simulink model "chaine_texte"  (R2023b)
settings: Solver=FixedStepDiscrete  StartTime=0.0  StopTime=(N/4 - 1)*4*Tb  FixedStep=4*Tb  RelTol=1e-3
values from neighbouring files (symbols this model uses):
  A = P.A    [parametres.m]    (also in partie2_1.m; partie2_5_q10.m = numel(unique(msg)); partie2_5_q11.m = numel(unique(seq)))
  Ac = A * sqrt(4/7)    [creer_chaine_hamming.m]
  graine = P.graine    [parametres.m]    (also in parametres_perso.m = mod(sum(c .* (1:numel(c)) * 31) + 7 * numel(c), 2^31 - 1); partie2_1.m)
  L = P.L    [parametres.m]    (also in partie2_1.m)
  sig2 = N0 * L / (2*Tb)    [parametres.m]    (also in partie3_q12.m = A^2 * L / (2 * 10^(EbN0dB/10)))
  Tb = 1    [parametres.m]    (also in partie2_1.m)
libraries: simulink x2
settings Model: Creator=e2507477  LastModifiedBy=e2507477

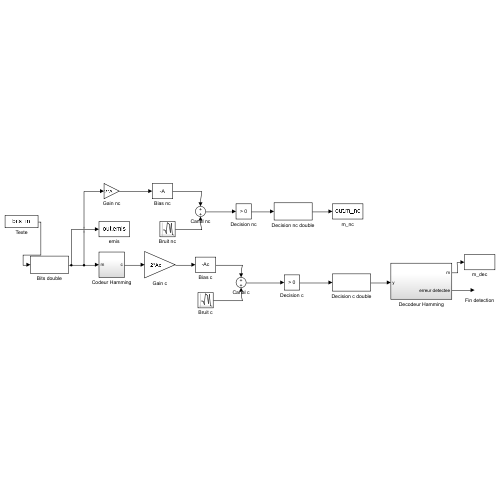
[thumbnail: Simulink's stored preview of the top-level diagram]
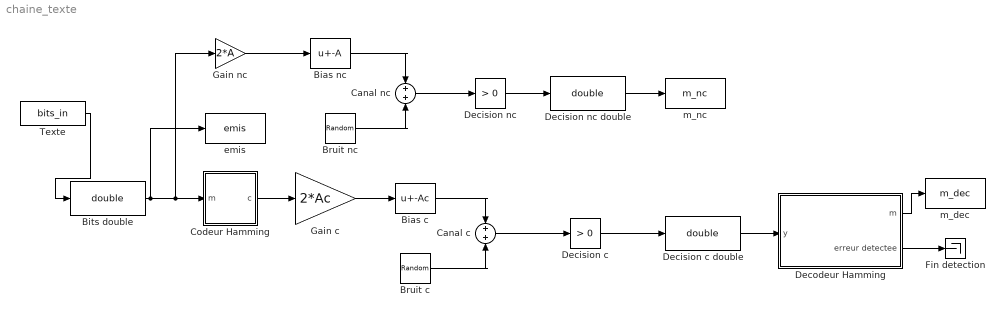
== system chaine_texte ==
  Bias c : Bias  Bias=-Ac  SaturateOnIntegerOverflow=off
  Bias nc : Bias  Bias=-A  SaturateOnIntegerOverflow=off
  Bits double : DataTypeConversion  OutDataTypeStr=double  SaturateOnIntegerOverflow=off  RndMeth=Floor
  Bruit c : RandomNumber  Mean=zeros(1,7)  Variance=sig2/L*ones(1,7)  Seed=round(graine) + 50000 + 7919*(0:6)  SampleTime=4*Tb
  Bruit nc : RandomNumber  Mean=zeros(1,4)  Variance=sig2/L*ones(1,4)  Seed=round(graine) + 90000 + 7919*(0:3)  SampleTime=4*Tb
  Canal c : Sum
  Canal nc : Sum
  Codeur Hamming : Subsystem
  Decision c : simulink/Logic and Bit Operations/Compare To Constant  relop=>  const=0  OutDataTypeStr=boolean
  Decision c double : DataTypeConversion  OutDataTypeStr=double  SaturateOnIntegerOverflow=off  RndMeth=Floor
  Decision nc : simulink/Logic and Bit Operations/Compare To Constant  relop=>  const=0  OutDataTypeStr=boolean
  Decision nc double : DataTypeConversion  OutDataTypeStr=double  SaturateOnIntegerOverflow=off  RndMeth=Floor
  Decodeur Hamming : Subsystem
  Fin detection : Terminator
  Gain c : Gain  Gain=2*Ac
  Gain nc : Gain  Gain=2*A
  Texte : FromWorkspace  VariableName=bits_in  SampleTime=4*Tb  Interpolate=off  OutputAfterFinalValue=Holding final value
  emis : ToWorkspace  VariableName=emis  SampleTime=-1
  m_dec : ToWorkspace  VariableName=m_dec  SampleTime=-1
  m_nc : ToWorkspace  VariableName=m_nc  SampleTime=-1
  wires:
  Bits double/1 -> Codeur Hamming/1(m), Gain nc/1, emis/1
  Bruit nc/1 -> Canal nc/2
  Decision nc/1 -> Decision nc double/1
  Bias nc/1 -> Canal nc/1
  Gain nc/1 -> Bias nc/1
  Codeur Hamming/1(c) -> Gain c/1
  Gain c/1 -> Bias c/1
  Canal nc/1 -> Decision nc/1
  Canal c/1 -> Decision c/1
  Bias c/1 -> Canal c/1
  Bruit c/1 -> Canal c/2
  Decision nc double/1 -> m_nc/1
  Decision c/1 -> Decision c double/1
  Decision c double/1 -> Decodeur Hamming/1(y)
  Decodeur Hamming/1(m) -> m_dec/1
  Decodeur Hamming/2(erreur detectee) -> Fin detection/1
  Texte/1 -> Bits double/1

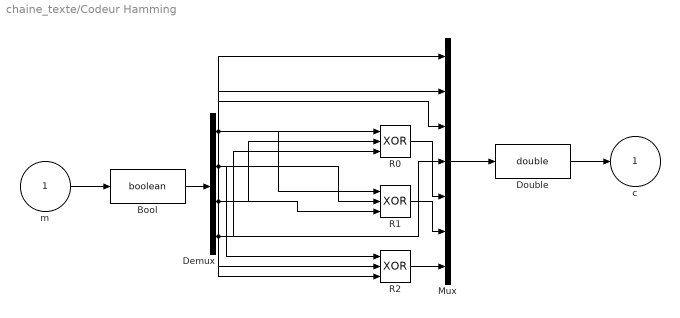
== system chaine_texte/Codeur Hamming ==
  m : Inport
  Bool : DataTypeConversion  OutDataTypeStr=boolean  SaturateOnIntegerOverflow=off  RndMeth=Floor
  Demux : Demux
  Double : DataTypeConversion  OutDataTypeStr=double  SaturateOnIntegerOverflow=off  RndMeth=Floor
  Mux : Mux  Inputs=7
  R0 : Logic  Operator=XOR  Inputs=3  AllPortsSameDT=off  OutDataTypeStr=boolean
  R1 : Logic  Operator=XOR  Inputs=3  AllPortsSameDT=off  OutDataTypeStr=boolean
  R2 : Logic  Operator=XOR  Inputs=3  AllPortsSameDT=off  OutDataTypeStr=boolean
  c : Outport
  wires:
  m/1 -> Bool/1
  Demux/2 -> Mux/2, R1/2, R2/1
  Demux/1 -> Mux/1, R0/1, R1/1
  Bool/1 -> Demux/1
  Demux/4 -> R0/3, R2/3, Mux/4
  Demux/3 -> Mux/3, R0/2, R1/3, R2/2
  R1/1 -> Mux/6
  R0/1 -> Mux/5
  R2/1 -> Mux/7
  Double/1 -> c/1
  Mux/1 -> Double/1

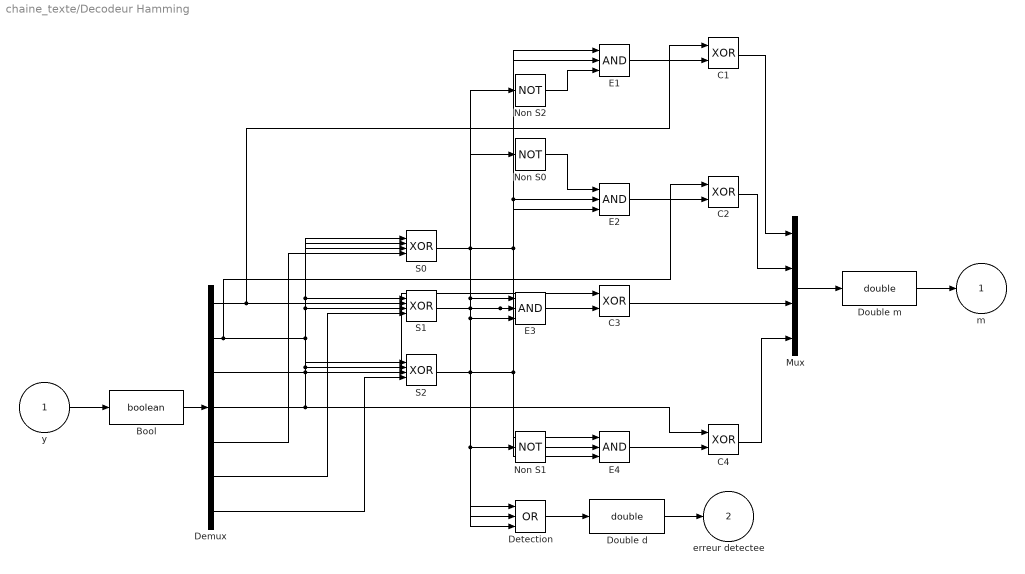
== system chaine_texte/Decodeur Hamming ==
  y : Inport
  Bool : DataTypeConversion  OutDataTypeStr=boolean  SaturateOnIntegerOverflow=off  RndMeth=Floor
  C{1..4} (4 alike) : Logic  Operator=XOR  AllPortsSameDT=off  OutDataTypeStr=boolean
  Demux : Demux  Outputs=7
  Detection : Logic  Operator=OR  Inputs=3  AllPortsSameDT=off  OutDataTypeStr=boolean
  Double d : DataTypeConversion  OutDataTypeStr=double  SaturateOnIntegerOverflow=off  RndMeth=Floor
  Double m : DataTypeConversion  OutDataTypeStr=double  SaturateOnIntegerOverflow=off  RndMeth=Floor
  E{1..4} (4 alike) : Logic  Inputs=3  AllPortsSameDT=off  OutDataTypeStr=boolean
  Mux : Mux
  Non S0 : Logic  Operator=NOT  AllPortsSameDT=off  OutDataTypeStr=boolean
  Non S1 : Logic  Operator=NOT  AllPortsSameDT=off  OutDataTypeStr=boolean
  Non S2 : Logic  Operator=NOT  AllPortsSameDT=off  OutDataTypeStr=boolean
  S0 : Logic  Operator=XOR  Inputs=4  AllPortsSameDT=off  OutDataTypeStr=boolean
  S1 : Logic  Operator=XOR  Inputs=4  AllPortsSameDT=off  OutDataTypeStr=boolean
  S2 : Logic  Operator=XOR  Inputs=4  AllPortsSameDT=off  OutDataTypeStr=boolean
  m : Outport
  erreur detectee : Outport  Port=2
  wires:
  Double m/1 -> m/1
  Mux/1 -> Double m/1
  C4/1 -> Mux/4
  C2/1 -> Mux/2
  C1/1 -> Mux/1
  Double d/1 -> erreur detectee/1
  E4/1 -> C4/2
  C3/1 -> Mux/3
  E2/1 -> C2/2
  E1/1 -> C1/2
  E3/1 -> C3/2
  Non S2/1 -> E1/3
  S2/1 -> Detection/3, Non S2/1, E3/3, E4/3, E2/3
  Demux/7 -> S2/4
  S0/1 -> Non S0/1, E4/1, E1/1, E3/1, Detection/1
  S1/1 -> E3/2, E2/2, E1/2, Detection/2, Non S1/1
  Demux/5 -> S0/4
  Detection/1 -> Double d/1
  Demux/1 -> C1/1, S1/1, S0/1
  Demux/3 -> C3/1, S2/2, S1/3, S0/2
  Demux/6 -> S1/4
  y/1 -> Bool/1
  Bool/1 -> Demux/1
  Demux/2 -> C2/1, S1/2, S2/1
  Non S0/1 -> E2/1
  Non S1/1 -> E4/2
  Demux/4 -> C4/1, S2/3, S0/3
